simulink model "zad6_sim"  (R2026a)
settings: Solver=VariableStepAuto  MaxStep=1e-3
settings Model: Creator=Michal_backup  LastModifiedBy=Michal_backup

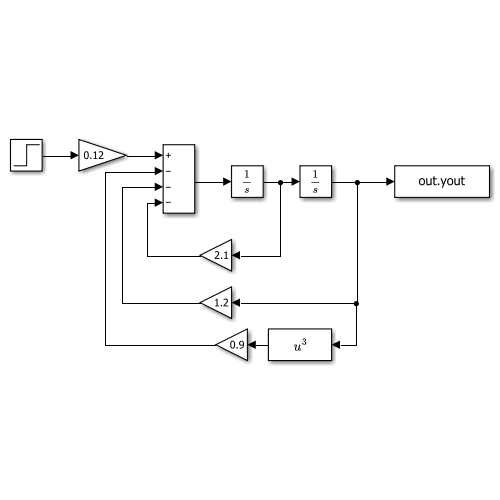
[thumbnail: Simulink's stored preview of the top-level diagram]
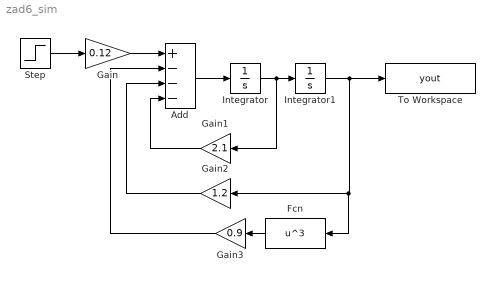
== system zad6_sim ==
  Add : Sum  Inputs=+---
  Fcn : Fcn  Expr=u^3
  Gain : Gain  Gain=0.12
  Gain1 : Gain  Gain=2.1
  Gain2 : Gain  Gain=1.2
  Gain3 : Gain  Gain=0.9
  Integrator : Integrator
  Integrator1 : Integrator
  Step : Step  FinalValue=U  SampleTime=0
  To Workspace : ToWorkspace  VariableName=yout  SaveFormat=Timeseries  SampleTime=-1
  wires:
  Step/1 -> Gain/1
  Gain/1 -> Add/1
  Add/1 -> Integrator/1
  Integrator/1 -> Gain1/1, Integrator1/1
  Gain1/1 -> Add/4
  Integrator1/1 -> To Workspace/1, Fcn/1, Gain2/1
  Gain2/1 -> Add/3
  Fcn/1 -> Gain3/1
  Gain3/1 -> Add/2
